simulink model "unmanned_aerial_vehicle_model"  (R2024b)
settings: Solver=ode4  StartTime=0.0  StopTime=10.0  FixedStep=0.01  RelTol=1e-3
undefined symbols (not defined in the file or in its folder): Kd_ang, Kd_pos, Kp_ang, Kp_pos
settings Model: Creator=meow  LastModifiedBy=meow

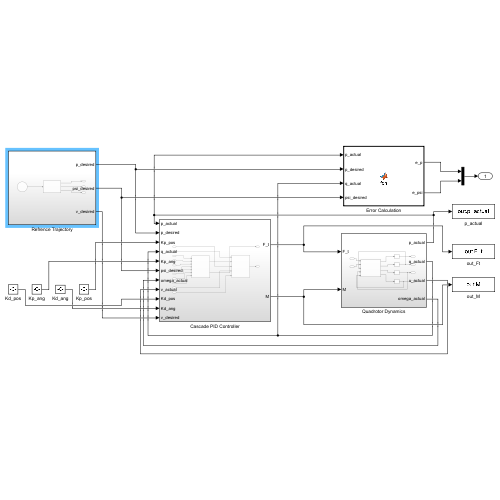
[thumbnail: Simulink's stored preview of the top-level diagram]
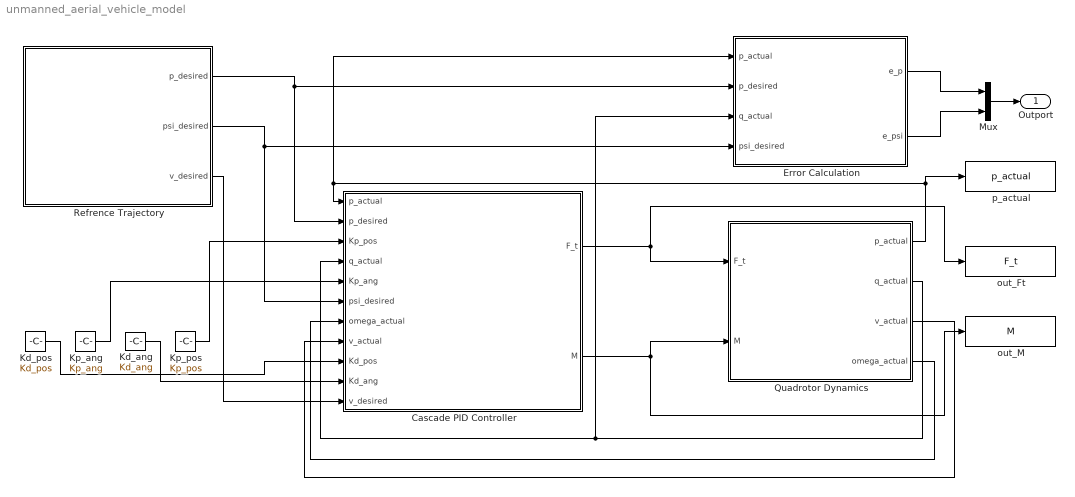
== system unmanned_aerial_vehicle_model ==
  Cascade PID Controller : Subsystem
  Error Calculation : MATLAB Function  TreatAsAtomicUnit=on
  Kd_ang : Constant  Value=Kd_ang
  Kd_pos : Constant  Value=Kd_pos
  Kp_ang : Constant  Value=Kp_ang
  Kp_pos : Constant  Value=Kp_pos
  Mux : Mux  Inputs=2
  Quadrotor Dynamics : Subsystem
  Refrence Trajectory : Subsystem
  out_Ft : ToWorkspace  VariableName=F_t  SampleTime=-1
  out_M : ToWorkspace  VariableName=M  SampleTime=-1
  p_actual : ToWorkspace  VariableName=p_actual  SampleTime=-1
  Outport : Outport
  wires:
  Refrence Trajectory/1(p_desired) -> Cascade PID Controller/2(p_desired), Error Calculation/2(p_desired)
  Cascade PID Controller/1(F_t) -> out_Ft/1, Quadrotor Dynamics/1(F_t)
  Cascade PID Controller/2(M) -> Quadrotor Dynamics/2(M), out_M/1
  Quadrotor Dynamics/1(p_actual) -> p_actual/1, Error Calculation/1(p_actual), Cascade PID Controller/1(p_actual)
  Quadrotor Dynamics/2(q_actual) -> Cascade PID Controller/4(q_actual), Error Calculation/3(q_actual)
  Kp_pos/1 -> Cascade PID Controller/3(Kp_pos)
  Kp_ang/1 -> Cascade PID Controller/5(Kp_ang)
  Refrence Trajectory/2(psi_desired) -> Cascade PID Controller/6(psi_desired), Error Calculation/4(psi_desired)
  Error Calculation/1(e_p) -> Mux/1
  Error Calculation/2(e_psi) -> Mux/2
  Mux/1 -> Outport/1
  Quadrotor Dynamics/3(v_actual) -> Cascade PID Controller/8(v_actual)
  Quadrotor Dynamics/4(omega_actual) -> Cascade PID Controller/7(omega_actual)
  Kd_pos/1 -> Cascade PID Controller/9(Kd_pos)
  Kd_ang/1 -> Cascade PID Controller/10(Kd_ang)
  Refrence Trajectory/3(v_desired) -> Cascade PID Controller/11(v_desired)

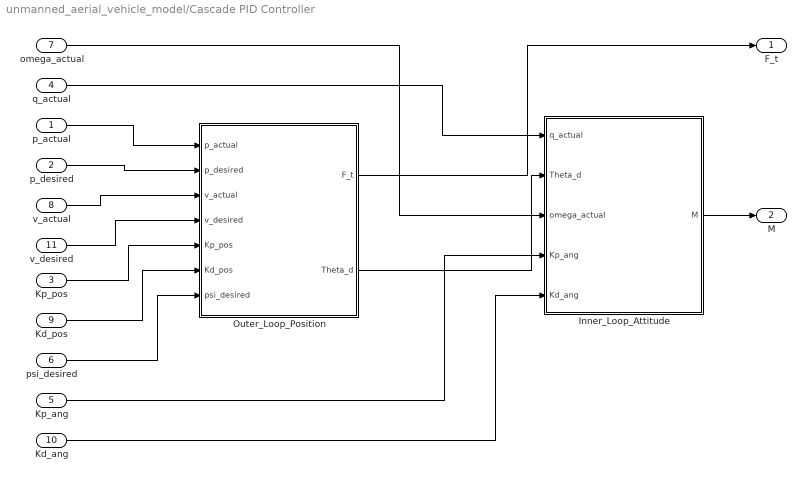
== system unmanned_aerial_vehicle_model/Cascade PID Controller ==
  p_actual : Inport
  p_desired : Inport  Port=2
  Kp_pos : Inport  Port=3
  q_actual : Inport  Port=4
  Kp_ang : Inport  Port=5
  psi_desired : Inport  Port=6
  omega_actual : Inport  Port=7
  v_actual : Inport  Port=8
  Kd_pos : Inport  Port=9
  Kd_ang : Inport  Port=10
  v_desired : Inport  Port=11
  Inner_Loop_Attitude : MATLAB Function  TreatAsAtomicUnit=on
  Outer_Loop_Position : MATLAB Function  TreatAsAtomicUnit=on
  F_t : Outport
  M : Outport  Port=2
  wires:
  Outer_Loop_Position/2(Theta_d) -> Inner_Loop_Attitude/2(Theta_d)
  p_actual/1 -> Outer_Loop_Position/1(p_actual)
  p_desired/1 -> Outer_Loop_Position/2(p_desired)
  Kp_pos/1 -> Outer_Loop_Position/5(Kp_pos)
  q_actual/1 -> Inner_Loop_Attitude/1(q_actual)
  Kp_ang/1 -> Inner_Loop_Attitude/4(Kp_ang)
  Outer_Loop_Position/1(F_t) -> F_t/1
  Inner_Loop_Attitude/1(M) -> M/1
  psi_desired/1 -> Outer_Loop_Position/7(psi_desired)
  v_actual/1 -> Outer_Loop_Position/3(v_actual)
  Kd_pos/1 -> Outer_Loop_Position/6(Kd_pos)
  omega_actual/1 -> Inner_Loop_Attitude/3(omega_actual)
  Kd_ang/1 -> Inner_Loop_Attitude/5(Kd_ang)
  v_desired/1 -> Outer_Loop_Position/4(v_desired)

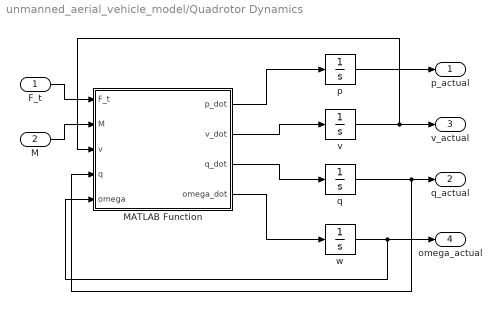
== system unmanned_aerial_vehicle_model/Quadrotor Dynamics ==
  F_t : Inport
  M : Inport  Port=2
  MATLAB Function : MATLAB Function  TreatAsAtomicUnit=on
  p : Integrator  InitialCondition=[0; 0; 0]
  q : Integrator  InitialCondition=[1; 0; 0; 0]
  v : Integrator  InitialCondition=[0; 0; 0]
  w : Integrator  InitialCondition=[0; 0; 0]
  p_actual : Outport
  q_actual : Outport  Port=2
  v_actual : Outport  Port=3
  omega_actual : Outport  Port=4
  wires:
  MATLAB Function/1(p_dot) -> p/1
  MATLAB Function/2(v_dot) -> v/1
  MATLAB Function/3(q_dot) -> q/1
  MATLAB Function/4(omega_dot) -> w/1
  v/1 -> MATLAB Function/3(v), v_actual/1
  w/1 -> MATLAB Function/5(omega), omega_actual/1
  F_t/1 -> MATLAB Function/1(F_t)
  M/1 -> MATLAB Function/2(M)
  p/1 -> p_actual/1
  q/1 -> MATLAB Function/4(q), q_actual/1

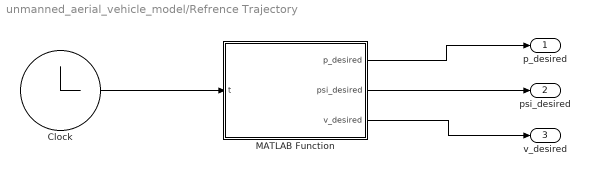
== system unmanned_aerial_vehicle_model/Refrence Trajectory ==
  Clock : Clock
  MATLAB Function : MATLAB Function  TreatAsAtomicUnit=on
  p_desired : Outport
  psi_desired : Outport  Port=2
  v_desired : Outport  Port=3
  wires:
  MATLAB Function/1(p_desired) -> p_desired/1
  MATLAB Function/2(psi_desired) -> psi_desired/1
  Clock/1 -> MATLAB Function/1(t)
  MATLAB Function/3(v_desired) -> v_desired/1

== matlab function unmanned_aerial_vehicle_model/Cascade PID Controller/Outer_Loop_Position ==
  data: p_actual input; F_t output; p_desired input; v_actual input; v_desired input; Kp_pos input; Kd_pos input; Theta_d output; psi_desired input
function [F_t, Theta_d] = fcn(p_actual, p_desired, v_actual, v_desired, Kp_pos, Kd_pos, psi_desired)
%% OUTER LOOP CASCADED PD CONTROLLER (POSITION -> ATTITUDE & THRUST)
% This function calculates the total required thrust (F_t) and the desired
% Euler angles (Theta_d = [roll; pitch; yaw]) to minimize the 3D spatial 
% trajectory tracking error.

%% 1. Input Sanitization
% Force all inputs to be column vectors to prevent matrix dimension 
% mismatch errors during continuous Simulink execution.
p_actual = p_actual(:); p_desired = p_desired(:); 
v_actual = v_actual(:); v_desired = v_desired(:);
Kp_pos = Kp_pos(:); Kd_pos = Kd_pos(:);

%% 2. Kinematic Error Calculation
% Calculate the proportional (position) and derivative (velocity) errors.
% Note: e_v utilizes the analytical derivative of the trajectory (v_desired)
% rather than assuming a static target, eliminating the "toilet bowl effect".
e_p = p_desired - p_actual;
e_v = v_desired - v_actual; 

%% 3. Desired Attitude (Spatial to Angular Mapping)
% Map the horizontal tracking errors to corresponding pitch and roll commands.
Theta_d = zeros(3,1);

% Pitch (Theta_d(2)): Controls X-axis movement.
% A positive X error requires a forward tilt (positive pitch).
Theta_d(2) = Kp_pos(1)*e_p(1) + Kd_pos(1)*e_v(1);

% Roll (Theta_d(1)): Controls Y-axis movement.
% A positive Y error (moving right) requires a rightward tilt (negative roll).
% The negative multiplier enforces correct spatial vectoring.
Theta_d(1) = -(Kp_pos(2)*e_p(2) + Kd_pos(2)*e_v(2));

% Yaw (Theta_d(3)): Direct passthrough of the reference heading.
Theta_d(3) = psi_desired;

%% 4. Attitude Saturation (Flight Envelope Protection)
% Hardcode physical limits to pitch and roll commands to prevent aerodynamic 
% stalling or catastrophic inversion (flipping) during aggressive tracking.
% Clamped to +/- 0.785 radians (45 degrees).
Theta_d(1) = max(min(Theta_d(1), 0.785), -0.785);
Theta_d(2) = max(min(Theta_d(2), 0.785), -0.785);

%% 5. Z-Axis Thrust & Altitude Compensation
% Calculate the baseline vertical thrust required to maintain altitude, 
% including the feedforward hover thrust (mg = 16.94 N).
F_t_ideal = Kp_pos(3)*e_p(3) + Kd_pos(3)*e_v(3) + 16.94;

% Compensate for lift-loss during maneuvers. When a quadrotor banks, the 
% thrust vector tilts, reducing the vertical component. Dividing by the 
% cosine of the commanded pitch and roll angles artificially boosts total 
% throttle to guarantee altitude is maintained through sharp curves.
F_t = F_t_ideal / (cos(Theta_d(1)) * cos(Theta_d(2)));

%% 6. Actuator Limits (Motor Saturation)
% Cap the absolute maximum thrust output to simulate physical motor limits 
% and prevent infinite mathematical spikes in the physics engine.
F_t = min(F_t, 40.0); 
end

== matlab function unmanned_aerial_vehicle_model/Quadrotor Dynamics/MATLAB Function ==
  data: F_t input; p_dot output; M input; v input; q input; omega input; v_dot output; q_dot output; omega_dot output
function [p_dot, v_dot, q_dot, omega_dot] = fcn(F_t, M, v, q, omega)
%% NONLINEAR QUADROTOR DYNAMICS (NEWTON-EULER EQUATIONS)
% This function calculates the state derivatives for a 6-DOF rigid body.
% It translates control efforts (Thrust and Torque) into linear and angular 
% accelerations, which Simulink's continuous solver will integrate into 
% velocity and position.

%% 1. Input Sanitization & Preallocation
% Enforce column vector dimensions to prevent matrix operation failures 
% during continuous-time ODE integration steps.
v = v(:); q = q(:); omega = omega(:); M = M(:);

p_dot = zeros(3,1);
v_dot = zeros(3,1);
q_dot = zeros(4,1);
omega_dot = zeros(3,1);

%% 2. Physical Constants (UAV Airframe Parameters)
m = 1.727; % Mass of the quadrotor (kg)
g = 9.81;  % Acceleration due to gravity (m/s^2)

% Inertia Tensor Matrix (kg*m^2)
% Assumes a symmetrical quadrotor body (off-diagonal products of inertia are zero)
J = diag([1.40e-5, 1.40e-5, 2.17e-5]);

%% 3. Attitude Representation (Body-to-Inertial Frame Mapping)
% Normalize the quaternion to enforce unit-length requirement. This prevents 
% mathematical drift caused by numerical errors during ODE integration.
q = q / norm(q);
q0 = q(1); q1 = q(2); q2 = q(3); q3 = q(4);

% Compute the Direction Cosine Matrix (Rotation Matrix) from Quaternions.
% This matrix rotates vectors from the UAV's Body Frame to the Inertial Frame.
R = [1-2*(q2^2+q3^2),  2*(q1*q2-q0*q3),  2*(q0*q2+q1*q3);
     2*(q1*q2+q0*q3),  1-2*(q1^2+q3^2),  2*(q2*q3-q0*q1);
     2*(q1*q3-q0*q2),  2*(q0*q1+q2*q3),  1-2*(q1^2+q2^2)];

%% 4. Translational Equations of Motion
% Translational Kinematics: The derivative of position is linear velocity.
p_dot = v;

% Translational Dynamics (Newton's Second Law: F = ma):
% Calculates linear acceleration in the Inertial Frame.
%   1. R * [0; 0; F_t] maps the total rotor thrust from the body's local Z-axis 
%      into global X/Y/Z vector components.
%   2. [0; 0; -m*g] applies the gravity vector pointing strictly downward.
v_dot = (1/m) * (R * [0; 0; F_t] + [0; 0; -m*g]);

%% 5. Rotational Equations of Motion
% Rotational Dynamics (Euler's Equation for Rigid Body Dynamics):
% Calculates angular acceleration (omega_dot) in the Body Frame.
% The 'cross(omega, J * omega)' term accounts for the nonlinear gyroscopic 
% coupling effects caused by the drone rotating in multiple axes simultaneously.
omega_dot = J \ (M - cross(omega, J * omega));

% Rotational Kinematics (Quaternion Derivative):
% Maps the body frame angular velocities (omega) into quaternion rates of change.
% This is the exact mathematical formulation preventing gimbal lock.
q_dot = 0.5 * [ q0, -q1, -q2, -q3;
                q1,  q0, -q3,  q2;
                q2,  q3,  q0, -q1;
                q3, -q2,  q1,  q0] * [0; omega];
end

== matlab function unmanned_aerial_vehicle_model/Cascade PID Controller/Inner_Loop_Attitude ==
  data: q_actual input; M output; Theta_d input; omega_actual input; Kp_ang input; Kd_ang input
function M = fcn(q_actual, Theta_d, omega_actual, Kp_ang, Kd_ang)
%% INNER LOOP ATTITUDE CONTROLLER (ATTITUDE -> TORQUE)
% This function calculates the 3D control torques (M = [tau_roll; tau_pitch; tau_yaw])
% required to rotate the quadrotor to the desired attitude commanded by the outer loop.
% It converts quaternion states to Euler angles and applies a PD control law.

%% 1. Input Sanitization
% Force all inputs to be column vectors to ensure element-wise matrix 
% operations execute correctly during continuous Simulink simulation.
q_actual = q_actual(:); Theta_d = Theta_d(:); omega_actual = omega_actual(:);
Kp_ang = Kp_ang(:); Kd_ang = Kd_ang(:);

%% 2. Quaternion Normalization
% The physics engine outputs orientations as quaternions to avoid gimbal lock.
% Numerical integration over time can cause the quaternion to drift from unit length.
% Normalizing guarantees it remains a valid rotation mathematical operator.
q_actual = q_actual / norm(q_actual);

% Extract scalar (q0) and vector (q1, q2, q3) components for standard ZYX conversion
q0 = q_actual(1); q1 = q_actual(2); q2 = q_actual(3); q3 = q_actual(4);

%% 3. Quaternion to Euler Angle Transformation
% Convert the actual orientation back into Euler angles (Roll, Pitch, Yaw)
% so they can be directly compared against the target angles (Theta_d).

% Roll (phi / X-axis rotation)
phi = atan2(2*(q0*q1 + q2*q3), 1 - 2*(q1^2 + q2^2));

% Pitch (theta / Y-axis rotation)
sinp = 2*(q0*q2 - q3*q1);
% Singularity Protection: Clamp the sine value to exactly [-1, 1] to prevent 
% complex number outputs from the asin() function due to floating-point errors.
sinp = max(-1, min(1, sinp));
theta = asin(sinp);

% Yaw (psi / Z-axis rotation)
psi = atan2(2*(q0*q3 + q1*q2), 1 - 2*(q2^2 + q3^2));

Theta_actual = [phi; theta; psi];

%% 4. Kinematic Error Calculation
% Calculate the proportional (angular) tracking error.
e_ang = Theta_d - Theta_actual;

% Calculate the derivative (angular velocity) tracking error.
% Note: The target angular velocity is assumed to be zero (0 - omega_actual). 
% This acts as pure rotational damping, actively braking the drone to 
% prevent overshoot as it reaches the target angle.
e_omega = -omega_actual; 

%% 5. Proportional-Derivative (PD) Control Law
% Compute the required restorative torque. 
% Proportional term pushes the drone toward the target angle.
% Derivative term resists the current spinning motion.
M = Kp_ang .* e_ang + Kd_ang .* e_omega;

%% 6. Actuator Saturation (Motor Limits)
% Hardcode physical torque limits. A micro-UAV motor physically cannot generate 
% infinite torque. Capping this at +/- 0.05 N-m prevents the mathematical model 
% from asking the motors to perform impossible instantaneous maneuvers, 
% preventing system instability and chatter.
M = max(min(M, 0.05), -0.05);

end

== matlab function unmanned_aerial_vehicle_model/Refrence Trajectory/MATLAB Function ==
  data: t input; p_desired output; psi_desired output; v_desired output
function [p_desired, psi_desired, v_desired] = fcn(t)
%% REFERENCE TRAJECTORY GENERATOR (FLIGHT DIRECTOR)
% This function acts as the kinematic flight director for the quadrotor. 
% It evaluates continuous-time parameterized equations to output the 
% target 3D spatial coordinates (p_desired), the feedforward velocity 
% vector (v_desired), and the desired heading (psi_desired).
%
% NOTE: The analytical velocity derivative (v_desired) is provided explicitly 
% to the outer-loop controller. Passing the true target velocity as a feedforward 
% term eliminates position-tracking phase lag during continuous, high-speed curves.

%% 1. Trajectory A: The Four-Leaf Clover (Aggressive Maneuver)
% Mathematical Basis: Cartesian conversion of the polar rose curve (r = 2*cos(2t)).
% Purpose: Evaluates transient stability and attitude saturation. The drone 
% must rapidly reverse its pitch and roll as it whips through the origin, 
% severely testing the controller's ability to prevent altitude drop.

%p_desired = [2*cos(t)*cos(2*t); 2*sin(t)*cos(2*t); 1];

% Analytical Derivative (Chain Rule applied to the spatial equations)
%v_x = 2 * (-sin(t)*cos(2*t) - 2*cos(t)*sin(2*t));
%v_y = 2 * (cos(t)*cos(2*t) - 2*sin(t)*sin(2*t));
%v_desired = [v_x; v_y; 0];

%psi_desired = 0;

%% 2. Trajectory B: The Ellipse (Baseline Circular Tracking)
% Mathematical Basis: Simple harmonic parametric equations.
% Purpose: Evaluates steady-state tracking accuracy. It tests the controller's 
% ability to smoothly maintain a constant horizontal velocity vector while 
% locked at a fixed altitude (Z=1).

%p_desired = [2*cos(t); 2*sin(t); 1];

% Analytical Derivative
%v_desired = [-2*sin(t); 2*cos(t); 0];

%psi_desired = 0;

%% 3. Trajectory C: The 3D Spiral (Altitude/Attitude Coordination)
% Mathematical Basis: Superposition of a horizontal circle and a linear Z-axis ramp.
% Purpose: Evaluates 3D spatial coupling. The controller must simultaneously 
% manage the bank angles required for circular X/Y flight while continuously 
% boosting total thrust to maintain a steady vertical climb rate.

% Spiral Position: Radius of 2m, climbing steadily at 0.1 m/s
p_desired = [2*cos(t); 2*sin(t); 0.1*t];

% Spiral Velocity: Constant horizontal speed, constant vertical climb
v_desired = [-2*sin(t); 2*cos(t); 0.1];

% Constant heading: The UAV nose remains locked to the global X-axis (0 rad)
psi_desired = 0;

end

== matlab function unmanned_aerial_vehicle_model/Error Calculation ==
  data: p_actual input; e_p output; p_desired input; e_psi output; q_actual input; psi_desired input
function [e_p, e_psi] = fcn(p_actual, p_desired, q_actual, psi_desired)
%% PERFORMANCE METRICS (TRACKING ERROR CALCULATION)
% This function calculates the scalar error metrics used by the optimization 
% algorithm (HBO) to evaluate the trajectory tracking performance of the 
% current control parameters.

%% 1. Translational Tracking Error
% Compute the L2 Euclidean norm of the 3D position difference. 
% This yields the absolute spatial distance (in meters) between the 
% quadrotor's center of mass and the analytical target point.
e_p = norm(p_actual - p_desired);

%% 2. Heading (Yaw) Extraction
% Extract the scalar (q0) and vector (q1, q2, q3) components from the 
% current attitude quaternion.
q0 = q_actual(1); q1 = q_actual(2); q2 = q_actual(3); q3 = q_actual(4);

% Convert the quaternion directly into the Euler yaw angle (psi) around the Z-axis.
% We isolate yaw here because pitch and roll are transient states used for 
% translation, whereas yaw is an independent heading objective.
psi_actual = atan2(2*(q0*q3 + q1*q2), 1 - 2*(q2^2 + q3^2));

%% 3. Rotational Tracking Error
% Calculate the absolute angular deviation (in radians) from the desired heading.
e_psi = abs(psi_actual - psi_desired);

end
